simulink model "aerodynamic_model_V1_2_Wrench"  (R2025b)
settings: Solver=ode4  StartTime=0.0  StopTime=0.3  FixedStep=Ts  RelTol=1e-3
InitFcn:
  | % Run initial_main.m first to load Ad,As,Tq_prop,Tq_mass,...
values from neighbouring files (symbols this model uses):
  alpha_du0_v_tail_L = trim_aero_ic.v_tail_L.alpha_du0    [initial_main_V1_1.m]
  alpha_du0_v_tail_R = trim_aero_ic.v_tail_R.alpha_du0    [initial_main_V1_1.m]
  alpha_du0_wing_L = trim_aero_ic.wing_L.alpha_du0    [initial_main_V1_1.m]
  alpha_du0_wing_R = trim_aero_ic.wing_R.alpha_du0    [initial_main_V1_1.m]
  As = sys_sd.A    [initial_main_V1_1.m]
  BladePitch_deg = 34    [initial_main_V1_1.m]
  Bs = sys_sd.B    [initial_main_V1_1.m]
  Cs = sys_sd.C    [initial_main_V1_1.m]
  ctrl_delta_lim_deg = strips.delta_lim_deg    [initial_main_V1_1.m]
  ctrl_map_aileron_L = aero.wing_L.map_aileron(:)    [initial_main_V1_1.m]
  ctrl_map_aileron_R = aero.wing_R.map_aileron(:)    [initial_main_V1_1.m]
  ctrl_map_tail_L = aero.v_tail_L.map_tail(:)    [initial_main_V1_1.m]
  ctrl_map_tail_R = aero.v_tail_R.map_tail(:)    [initial_main_V1_1.m]
  Ds = sys_sd.D    [initial_main_V1_1.m]
  I_cg_b = R_sb * I_cg_m * R_sb.'    [aeroelastic.m]    (also in initial_main_V1_1.m = grav.I_cg_b)
  I_cg_b_inv = R_sb * I_cg_m_inv * R_sb.'    [aeroelastic.m]    (also in initial_main_V1_1.m = grav.I_cg_b_inv)
  m_node = zeros(n_id, 1)    [aeroelastic.m]    (also in generate_pullup_load_cloud.m = evalin('base', 'm_node(:)'); initial_main_V1_1.m = nodal.m_node)
  m_total_kg = evalin('base', 'm_total_kg')    [generate_pullup_load_cloud.m]    (also in initial_main_V1_1.m = grav.m_total_kg)
  n_modes = size(Phi, 2)    [aeroelastic.m]    (also in initial_main_V1_1.m = n_rigid + n_elastic)
  ones_1_tail = ones(1, size(r_cg2ac_b_v_tail_L, 2))    [initial_main_V1_1.m]
  ones_1_wing = ones(1, size(r_cg2ac_b_wing_L, 2))    [initial_main_V1_1.m]
  Phi = evalin('base', 'Phi')    [generate_pullup_load_cloud.m]    (also in initial_main_V1_1.m = strips.Phi)
  polar_alpha_deg = polar.alpha_deg(:).'    [initial_main_V1_1.m]
  polar_CD = polar.CD(:).'    [initial_main_V1_1.m]
  polar_CDp = polar.CDp(:).'    [initial_main_V1_1.m]
  polar_CL = polar.CL(:).'    [initial_main_V1_1.m]
  polar_CM = polar.CM(:).'    [initial_main_V1_1.m]
  r_cg2ac_b_v_tail_L = R_sb * aero.v_tail_L.r_ac_s    [initial_main_V1_1.m]
  r_cg2ac_b_v_tail_R = R_sb * aero.v_tail_R.r_ac_s    [initial_main_V1_1.m]
  r_cg2ac_b_wing_L = R_sb * aero.wing_L.r_ac_s    [initial_main_V1_1.m]
  r_cg2ac_b_wing_R = R_sb * aero.wing_R.r_ac_s    [initial_main_V1_1.m]
  r_cg2kink_b = eng.r_cg2kink_b    [initial_main_V1_1.m]
  r_cg2node_b = aeroelastic.node_arms(nodes, 'R_sb', R_sb).r_cg2node_b    [initial_main_V1_1.m]
  surface_nodes = aeroelastic.surface_load_nodes(nodes)    [initial_main_V1_1.m]
  T_aero2W = aeroelastic.wing_aileron_to_W(strips).T    [initial_main_V1_1.m]
  T_prop2W = load_maps.T_prop2W    [initial_main_V1_1.m]
  Tq_mass = load_maps.Tq_mass    [initial_main_V1_1.m]
  trim_Attitude_rad0 = trim_default.Attitude_rad0    [initial_main_V1_1.m]
  trim_Omega_b0 = trim_default.Omega_b0    [initial_main_V1_1.m]
  trim_Position0 = trim_default.Position0    [initial_main_V1_1.m]
  trim_Velocity_b0 = trim_default.Velocity_b0    [initial_main_V1_1.m]
  Ts = 0.001    [initial_main_V1_1.m]
  U = 55    [initial_main_V1_1.m]
  v_tail_cant_rad = deg2rad(v_tail_cant_deg)    [initial_main_V1_1.m]
  W_mass_g = grav.W_mass    [initial_main_V1_1.m]
  x0_structure = trim_default.x0_structure    [initial_main_V1_1.m]
  x0_wagner_v_tail_L = trim_aero_ic.v_tail_L.x0_wagner    [initial_main_V1_1.m]
  x0_wagner_v_tail_R = trim_aero_ic.v_tail_R.x0_wagner    [initial_main_V1_1.m]
  x0_wagner_wing_L = trim_aero_ic.wing_L.x0_wagner    [initial_main_V1_1.m]
  x0_wagner_wing_R = trim_aero_ic.wing_R.x0_wagner    [initial_main_V1_1.m]
undefined symbols (not defined in the file or in its folder): Ad_v_tail_L, Ad_v_tail_R, Ad_wing_L, Ad_wing_R, Bd_v_tail_L, Bd_v_tail_R, Bd_wing_L, Bd_wing_R, c_over_2U_v_tail_L, c_over_2U_v_tail_R, c_over_2U_wing_L, c_over_2U_wing_R, Cd_v_tail_L, Cd_v_tail_R, Cd_wing_L, Cd_wing_R, Dd_v_tail_L, Dd_v_tail_R, Dd_wing_L, Dd_wing_R, G_du_v_tail_L, G_du_v_tail_R, G_du_wing_L, G_du_wing_R, polar_aileron_alpha_deg, polar_aileron_dCD, polar_aileron_dCL, polar_aileron_dCM, polar_aileron_delta_deg, polar_ruddervator_alpha_deg, polar_ruddervator_dCD, polar_ruddervator_dCL, polar_ruddervator_dCM, polar_ruddervator_delta_deg, qS_strip_v_tail_L, qS_strip_v_tail_R, qS_strip_wing_L, qS_strip_wing_R, qSc_strip_v_tail_L, qSc_strip_v_tail_R, qSc_strip_wing_L, qSc_strip_wing_R, T_m2b_v_tail_L, T_m2b_v_tail_R, T_m2b_wing_L, T_m2b_wing_R, T_m2h_v_tail_L, T_m2h_v_tail_R, T_m2h_wing_L, T_m2h_wing_R, Tq_CM_v_tail_L, Tq_CM_v_tail_R, Tq_CM_wing_L, Tq_CM_wing_R, Tq_D_v_tail_L, Tq_D_v_tail_R, Tq_D_wing_L, Tq_D_wing_R, Tq_v_tail_L, Tq_v_tail_R ... (+2)
libraries: Prop_gryo x12, matrix_library x2
(part 2 of 6)

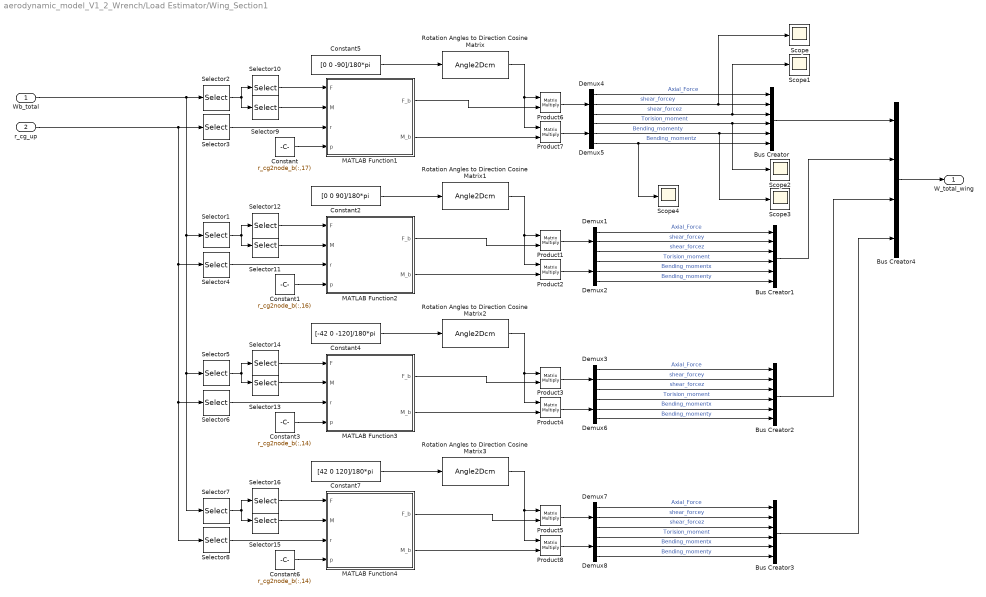
== system aerodynamic_model_V1_2_Wrench/Load Estimator/Wing_Section1 ==
  Wb_total : Inport
  r_cg_up : Inport  Port=2
  Bus Creator{,1..3} (4 alike) : BusCreator  Inputs=6
  Bus Creator4 : BusCreator  Inputs=4
  Constant : Constant  Value=r_cg2node_b(:,17)
  Constant1 : Constant  Value=r_cg2node_b(:,16)
  Constant2 : Constant  Value=[0 0 90]/180*pi
  Constant3 : Constant  Value=r_cg2node_b(:,14)
  Constant4 : Constant  Value=[-42 0 -120]/180*pi
  Constant5 : Constant  Value=[0 0 -90]/180*pi
  Constant6 : Constant  Value=r_cg2node_b(:,14)
  Constant7 : Constant  Value=[42 0 120]/180*pi
  Demux{1..8} (8 alike) : Demux  Outputs=3
  MATLAB Function1 : MATLAB Function  TreatAsAtomicUnit=on
  MATLAB Function2 : MATLAB Function  TreatAsAtomicUnit=on
  MATLAB Function3 : MATLAB Function  TreatAsAtomicUnit=on
  MATLAB Function4 : MATLAB Function  TreatAsAtomicUnit=on
  Product{1..8} (8 alike) : Product  Multiplication=Matrix(*)
  Rotation Angles to Direction Cosine Matrix{,1..3} (4 alike) : Angle2Dcm  rotationOrder=XYZ
      settings: AttributesFormatString=Rotation Order: %<rotationOrder>
  Scope{,1..4} (5 alike) : Scope
      Scope settings: ActiveDisplayYMinimum=-701.70070889117164  ActiveDisplayYMaximum=2692.587568384824  DataLoggingVariableName=ScopeData3
      Scope1 settings: ActiveDisplayYMinimum=-5860.8762190817188  ActiveDisplayYMaximum=-5388.1734134448989  DataLoggingVariableName=ScopeData4
      Scope2 settings: ActiveDisplayYMinimum=-1  ActiveDisplayYMaximum=1  DataLoggingVariableName=ScopeData5
      Scope3 settings: ActiveDisplayYMinimum=-45751.57172735683  ActiveDisplayYMaximum=65131.541259439364  DataLoggingVariableName=ScopeData6
      Scope4 settings: ActiveDisplayYMinimum=-1  ActiveDisplayYMaximum=1  DataLoggingVariableName=ScopeData7
  Selector1 : Selector  NumberOfDimensions=2  InputPortWidth=3  IndexOptions=Select all,Index vector (dialog)  Indices=[1:6],[surface_nodes.wing_R.node_id]  OutputSizes=1,1
  Selector{10,12,14,16} (4 alike) : Selector  NumberOfDimensions=2  InputPortWidth=3  IndexOptions=Index vector (dialog),Select all  Indices=[1:3],[surface_nodes.wing_R.node_id]  OutputSizes=1,1
  Selector{9,11,13,15} (4 alike) : Selector  NumberOfDimensions=2  InputPortWidth=3  IndexOptions=Index vector (dialog),Select all  Indices=[4:6],[surface_nodes.wing_R.node_id]  OutputSizes=1,1
  Selector2 : Selector  NumberOfDimensions=2  InputPortWidth=3  IndexOptions=Select all,Index vector (dialog)  Indices=[1:6],[surface_nodes.wing_L.node_id]  OutputSizes=1,1
  Selector3 : Selector  NumberOfDimensions=2  InputPortWidth=3  IndexOptions=Select all,Index vector (dialog)  Indices=[1:6],[surface_nodes.wing_L.node_id]  OutputSizes=1,1
  Selector4 : Selector  NumberOfDimensions=2  InputPortWidth=3  IndexOptions=Select all,Index vector (dialog)  Indices=[1:6],[surface_nodes.wing_R.node_id]  OutputSizes=1,1
  Selector5 : Selector  NumberOfDimensions=2  InputPortWidth=3  IndexOptions=Select all,Index vector (dialog)  Indices=[1:6],[surface_nodes.v_tail_L.node_id]  OutputSizes=1,1
  Selector6 : Selector  NumberOfDimensions=2  InputPortWidth=3  IndexOptions=Select all,Index vector (dialog)  Indices=[1:6],[surface_nodes.v_tail_L.node_id]  OutputSizes=1,1
  Selector7 : Selector  NumberOfDimensions=2  InputPortWidth=3  IndexOptions=Select all,Index vector (dialog)  Indices=[1:6],[surface_nodes.v_tail_R.node_id]  OutputSizes=1,1
  Selector8 : Selector  NumberOfDimensions=2  InputPortWidth=3  IndexOptions=Select all,Index vector (dialog)  Indices=[1:6],[surface_nodes.v_tail_R.node_id]  OutputSizes=1,1
  W_total_wing : Outport
  wires:
  Selector9/1 -> MATLAB Function1/2(M)
  Selector10/1 -> MATLAB Function1/1(F)
  Selector2/1 -> Selector9/1, Selector10/1
  Constant/1 -> MATLAB Function1/4(p)
  Bus Creator4/1 -> W_total_wing/1
  Bus Creator3/1 -> Bus Creator4/4
  Bus Creator2/1 -> Bus Creator4/3
  Bus Creator1/1 -> Bus Creator4/2
  Bus Creator/1 -> Bus Creator4/1
  Demux7/1 -> Bus Creator3/1  "Axial_Force"
  Demux8/1 -> Bus Creator3/4  "Torision_moment"
  Demux7/2 -> Bus Creator3/2  "shear_forcey"
  Product8/1 -> Demux8/1
  Demux8/2 -> Bus Creator3/5  "Bending_momentx"
  Demux8/3 -> Bus Creator3/6  "Bending_momenty"
  Demux7/3 -> Bus Creator3/3  "shear_forcez"
  Product5/1 -> Demux7/1
  Product3/1 -> Demux3/1
  Product4/1 -> Demux6/1
  Demux3/2 -> Bus Creator2/2  "shear_forcey"
  Demux6/2 -> Bus Creator2/5  "Bending_momentx"
  Demux3/1 -> Bus Creator2/1  "Axial_Force"
  Demux3/3 -> Bus Creator2/3  "shear_forcez"
  Demux6/3 -> Bus Creator2/6  "Bending_momenty"
  Demux6/1 -> Bus Creator2/4  "Torision_moment"
  Demux2/1 -> Bus Creator1/4  "Torision_moment"
  Demux1/3 -> Bus Creator1/3  "shear_forcez"
  Demux2/3 -> Bus Creator1/6  "Bending_momenty"
  Demux1/2 -> Bus Creator1/2  "shear_forcey"
  Demux2/2 -> Bus Creator1/5  "Bending_momentx"
  Demux1/1 -> Bus Creator1/1  "Axial_Force"
  Demux4/1 -> Bus Creator/1  "Axial_Force"
  Demux5/3 -> Bus Creator/6, Scope4/1  "Bending_momentz"
  Demux5/2 -> Bus Creator/5, Scope3/1  "Bending_momenty"
  Demux5/1 -> Bus Creator/4, Scope2/1  "Torision_moment"
  Demux4/3 -> Bus Creator/3, Scope1/1  "shear_forcez"
  Demux4/2 -> Bus Creator/2, Scope/1  "shear_forcey"
  Selector16/1 -> MATLAB Function4/1(F)
  Selector15/1 -> MATLAB Function4/2(M)
  Selector7/1 -> Selector16/1, Selector15/1
  Selector14/1 -> MATLAB Function3/1(F)
  Selector13/1 -> MATLAB Function3/2(M)
  Selector5/1 -> Selector14/1, Selector13/1
  Selector1/1 -> Selector12/1, Selector11/1
  Selector11/1 -> MATLAB Function2/2(M)
  Selector12/1 -> MATLAB Function2/1(F)
  Product2/1 -> Demux2/1
  Product1/1 -> Demux1/1
  Product7/1 -> Demux5/1
  Product6/1 -> Demux4/1
  Constant7/1 -> Rotation Angles to Direction Cosine Matrix3/1
  MATLAB Function4/1(F_b) -> Product5/2
  Selector8/1 -> MATLAB Function4/3(r)
  Constant6/1 -> MATLAB Function4/4(p)
  Rotation Angles to Direction Cosine Matrix3/1 -> Product8/1, Product5/1
  MATLAB Function4/2(M_b) -> Product8/2
  r_cg_up/1 -> Selector3/1, Selector4/1, Selector6/1, Selector8/1
  Wb_total/1 -> Selector2/1, Selector7/1, Selector5/1, Selector1/1
  MATLAB Function3/2(M_b) -> Product4/2
  Rotation Angles to Direction Cosine Matrix2/1 -> Product3/1, Product4/1
  Constant3/1 -> MATLAB Function3/4(p)
  Selector6/1 -> MATLAB Function3/3(r)
  MATLAB Function3/1(F_b) -> Product3/2
  Constant4/1 -> Rotation Angles to Direction Cosine Matrix2/1
  Constant2/1 -> Rotation Angles to Direction Cosine Matrix1/1
  MATLAB Function2/1(F_b) -> Product1/2
  Selector4/1 -> MATLAB Function2/3(r)
  Constant1/1 -> MATLAB Function2/4(p)
  Rotation Angles to Direction Cosine Matrix1/1 -> Product2/1, Product1/1
  MATLAB Function2/2(M_b) -> Product2/2
  MATLAB Function1/2(M_b) -> Product7/2
  Rotation Angles to Direction Cosine Matrix/1 -> Product6/1, Product7/1
  Selector3/1 -> MATLAB Function1/3(r)
  MATLAB Function1/1(F_b) -> Product6/2
  Constant5/1 -> Rotation Angles to Direction Cosine Matrix/1

== system aerodynamic_model_V1_2_Wrench/Propulsion Dynamics/Subsystem8 ==
  In1 : Inport
  In2 : Inport  Port=2
  Vb : Inport  Port=3
  Omegab : Inport  Port=4
  BladePitchAngle_DEG : Inport  Port=5
  RPS : Inport  Port=6
  +Cant : Constant  Value=7/180*pi
  -Cant1 : Constant  Value=-7/180*pi
  -Cant10 : Constant  Value=r_cg2kink_b(:,8)
  -Cant11 : Constant  Value=-0.6
  -Cant2 : Constant  Value=0.6
  -Cant3 : Constant  Value=r_cg2kink_b(:,1)
  -Cant4 : Constant  Value=r_cg2kink_b(:,2)
  -Cant5 : Constant  Value=r_cg2kink_b(:,3)
  -Cant6 : Constant  Value=r_cg2kink_b(:,4)
  -Cant7 : Constant  Value=r_cg2kink_b(:,5)
  -Cant8 : Constant  Value=r_cg2kink_b(:,6)
  -Cant9 : Constant  Value=r_cg2kink_b(:,7)
  Demux : Demux  Outputs=8
  Demux1 : Demux  Outputs=8
  Demux2 : Demux  Outputs=8
  Prop1 : Prop_gryo/Prop1  SystemSampleTime=-1  VariantActivationTime=update diagram  EmptyChoice=off  PassThrough=off  PassThroughVariantControl=(default)  EmptyChoiceVariantControl=(default)  AllowFlexibleInterface=on  Latency=0  AutoFrameSizeCalculation=off
  Prop2 : Prop_gryo/Prop2  SystemSampleTime=-1  VariantActivationTime=update diagram  EmptyChoice=off  PassThrough=off  PassThroughVariantControl=(default)  EmptyChoiceVariantControl=(default)  AllowFlexibleInterface=on  Latency=0  AutoFrameSizeCalculation=off
  Prop3 : Prop_gryo/Prop3  SystemSampleTime=-1  VariantActivationTime=update diagram  EmptyChoice=off  PassThrough=off  PassThroughVariantControl=(default)  EmptyChoiceVariantControl=(default)  AllowFlexibleInterface=on  Latency=0  AutoFrameSizeCalculation=off
  Prop4 : Prop_gryo/Prop4  SystemSampleTime=-1  VariantActivationTime=update diagram  EmptyChoice=off  PassThrough=off  PassThroughVariantControl=(default)  EmptyChoiceVariantControl=(default)  AllowFlexibleInterface=on  Latency=0  AutoFrameSizeCalculation=off
  Prop5 : Prop_gryo/Prop5  SystemSampleTime=-1  VariantActivationTime=update diagram  EmptyChoice=off  PassThrough=off  PassThroughVariantControl=(default)  EmptyChoiceVariantControl=(default)  AllowFlexibleInterface=on  Latency=0  AutoFrameSizeCalculation=off
  Prop6 : Prop_gryo/Prop6  SystemSampleTime=-1  VariantActivationTime=update diagram  EmptyChoice=off  PassThrough=off  PassThroughVariantControl=(default)  EmptyChoiceVariantControl=(default)  AllowFlexibleInterface=on  Latency=0  AutoFrameSizeCalculation=off
  Prop7 : Prop_gryo/Prop7  SystemSampleTime=-1  VariantActivationTime=update diagram  EmptyChoice=off  PassThrough=off  PassThroughVariantControl=(default)  EmptyChoiceVariantControl=(default)  AllowFlexibleInterface=on  Latency=0  AutoFrameSizeCalculation=off
  Prop8 : Prop_gryo/Prop8  SystemSampleTime=-1  VariantActivationTime=update diagram  EmptyChoice=off  PassThrough=off  PassThroughVariantControl=(default)  EmptyChoiceVariantControl=(default)  AllowFlexibleInterface=on  Latency=0  AutoFrameSizeCalculation=off
  Out Bus Element : Outport  PortName=Prop  Element=signal1
  Out Bus Element1 : Outport  PortName=Prop  Element=signal2
  Out Bus Element2 : Outport  PortName=Prop  Element=signal3
  Out Bus Element3 : Outport  PortName=Prop  Element=signal4
  Out Bus Element4 : Outport  PortName=Prop  Element=signal5
  Out Bus Element5 : Outport  PortName=Prop  Element=signal6
  Out Bus Element6 : Outport  PortName=Prop  Element=signal7
  Out Bus Element7 : Outport  PortName=Prop  Element=signal8
  wires:
  In2/1 -> Demux1/1
  -Cant7/1 -> Prop5/4
  Vb/1 -> Prop5/2, Prop1/2, Prop4/2, Prop8/2, Prop7/3, Prop3/3, Prop6/3, Prop2/3
  Demux/7 -> Prop7/2
  Omegab/1 -> Prop5/3, Prop1/3, Prop4/3, Prop8/3, Prop7/4, Prop3/4, Prop6/4, Prop2/4
  Demux1/3 -> Prop3/6
  Demux1/6 -> Prop6/6
  -Cant8/1 -> Prop6/5
  -Cant1/1 -> Prop5/1, Prop1/1, Prop6/1, Prop2/1
  BladePitchAngle_DEG/1 -> Prop6/9, Prop2/9, Prop3/9, Prop7/9
  -Cant6/1 -> Prop4/4
  Demux1/2 -> Prop2/6
  Demux/6 -> Prop6/2
  -Cant5/1 -> Prop3/5
  -Cant4/1 -> Prop2/5
  +Cant/1 -> Prop4/1, Prop8/1, Prop3/1, Prop7/1
  -Cant3/1 -> Prop1/4
  Demux/2 -> Prop2/2
  -Cant10/1 -> Prop8/4
  Demux1/7 -> Prop7/6
  -Cant9/1 -> Prop7/5
  Demux/3 -> Prop3/2
  In1/1 -> Demux/1
  Prop1/1 -> Out Bus Element/1
  Prop2/1 -> Out Bus Element1/1
  RPS/1 -> Demux2/1
  Demux2/1 -> Prop1/6
  Demux2/2 -> Prop2/8
  Demux2/3 -> Prop3/8
  Demux2/4 -> Prop4/6
  Demux2/5 -> Prop5/6
  Demux2/6 -> Prop6/8
  Demux2/7 -> Prop7/8
  Demux2/8 -> Prop8/6
  Prop3/1 -> Out Bus Element2/1
  Prop4/1 -> Out Bus Element3/1
  Prop5/1 -> Out Bus Element4/1
  Prop6/1 -> Out Bus Element5/1
  Prop8/1 -> Out Bus Element7/1
  Prop7/1 -> Out Bus Element6/1
  -Cant2/1 -> Prop2/7, Prop3/7, Prop4/5, Prop1/5
  -Cant11/1 -> Prop6/7, Prop7/7, Prop8/5, Prop5/5

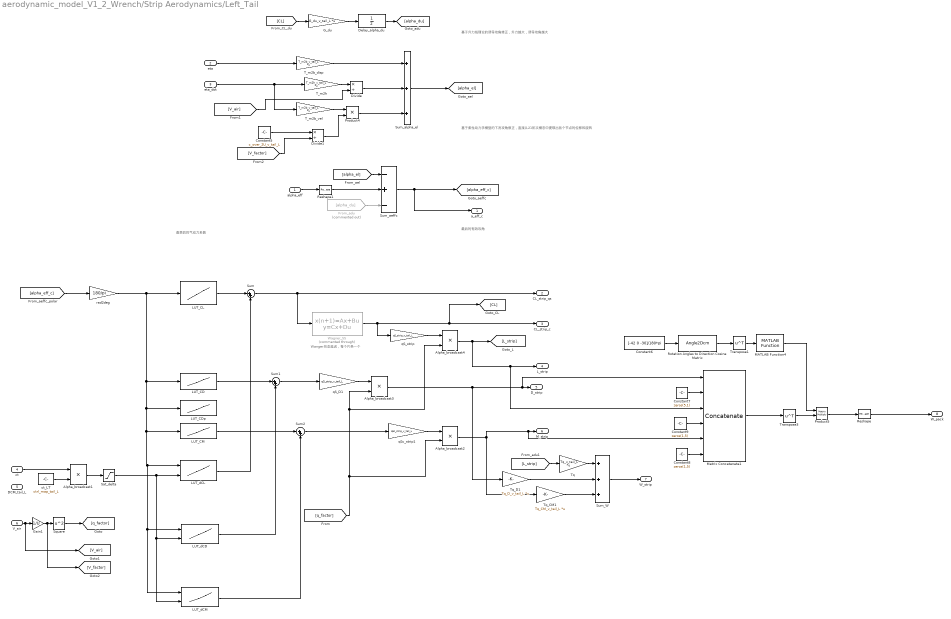
== system aerodynamic_model_V1_2_Wrench/Strip Aerodynamics/Left_Tail ==
  note: 基于升力线理论的诱导攻角修正，升力越大，诱导攻角越大
  note: 基于柔性动力学模型的下洗攻角修正，直接从21阶次模态中提取出各个节点的位移和旋转
  note: 最后的有效攻角
  note: 查表后的气动力系数
  note: Wanger状态延迟，每个片条一个
  alpha_eff : Inport
  eta : Inport  Port=2
  eta_dot : Inport  Port=3
  ct : Inport  Port=4
  DCM_tail_L : Inport  Port=5
  V_air : Inport  Port=6
  Alpha_broadcast{1..4} (4 alike) : Product  Inputs=**
  Constant5 : Constant  Value=c_over_2U_v_tail_L
  Constant6 : Constant  Value=[-42 0 -30]/180*pi
  Constant7 : Constant  Value=zeros(5,1)
  Constant8 : Constant  Value=zeros(1,5)
  Constant9 : Constant  Value=zeros(1,5)
  Delay_alpha_du : UnitDelay  InitialCondition=alpha_du0_v_tail_L  SampleTime=Ts  HasFrameUpgradeWarning=on
  Divide : Product  Inputs=*/
  Divide1 : Product  Inputs=*/
  From_adu : From  Commented=on  GotoTag=alpha_du
  G_du : Gain  Gain=G_du_v_tail_L  Multiplication=Matrix(K*u)
  Gain1 : Gain  Gain=1/U
  LUT_CD : Lookup_n-D  NumberOfTableDimensions=1  BreakpointsForDimension1=polar_alpha_deg  BreakpointsForDimension3=[5, 7]  Table=polar_CD  ExtrapMethod=Clip  InternalRulePriority=Speed  RndMeth=Simplest
  LUT_CDp : Lookup_n-D  NumberOfTableDimensions=1  BreakpointsForDimension1=polar_alpha_deg  BreakpointsForDimension3=[5, 7]  Table=polar_CDp  ExtrapMethod=Clip  InternalRulePriority=Speed  RndMeth=Simplest
  LUT_CL : Lookup_n-D  NumberOfTableDimensions=1  BreakpointsForDimension1=polar_alpha_deg  BreakpointsForDimension3=[5, 7]  Table=polar_CL  ExtrapMethod=Clip  InternalRulePriority=Speed  RndMeth=Simplest
  LUT_CM : Lookup_n-D  NumberOfTableDimensions=1  BreakpointsForDimension1=polar_alpha_deg  BreakpointsForDimension3=[5, 7]  Table=polar_CM  ExtrapMethod=Clip  InternalRulePriority=Speed  RndMeth=Simplest
  LUT_dCD : Lookup_n-D  BreakpointsForDimension1=polar_ruddervator_alpha_deg  BreakpointsForDimension2=polar_ruddervator_delta_deg  BreakpointsForDimension3=[5, 7]  Table=polar_ruddervator_dCD  ExtrapMethod=Clip  InternalRulePriority=Speed  RndMeth=Simplest
      settings: InputPortMap=u0,u1
  LUT_dCL : Lookup_n-D  BreakpointsForDimension1=polar_ruddervator_alpha_deg  BreakpointsForDimension2=polar_ruddervator_delta_deg  BreakpointsForDimension3=[5, 7]  Table=polar_ruddervator_dCL  ExtrapMethod=Clip  InternalRulePriority=Speed  RndMeth=Simplest
      settings: InputPortMap=u0,u1
  LUT_dCM : Lookup_n-D  BreakpointsForDimension1=polar_ruddervator_alpha_deg  BreakpointsForDimension2=polar_ruddervator_delta_deg  BreakpointsForDimension3=[5, 7]  Table=polar_ruddervator_dCM  ExtrapMethod=Clip  InternalRulePriority=Speed  RndMeth=Simplest
      settings: InputPortMap=u0,u1
  MATLAB Function4 : Prop_gryo/Prop1/MATLAB Function  SystemSampleTime=-1  VariantActivationTime=update diagram  EmptyChoice=off  PassThrough=off  PassThroughVariantControl=(default)  EmptyChoiceVariantControl=(default)  AllowFlexibleInterface=on  Latency=0  AutoFrameSizeCalculation=off
  Matrix Concatenate1 : Concatenate  NumInputs=6  Mode=Multidimensional array  ConcatenateDimension=2
  Product4 : Product
  Product5 : Product  Multiplication=Matrix(*)
  Reshape : Reshape
  Reshape1 : Reshape
  Rotation Angles to Direction Cosine Matrix : Angle2Dcm  rotationOrder=XYZ
      settings: AttributesFormatString=Rotation Order: %<rotationOrder>
  Sat_delta : Saturate  UpperLimit=ctrl_delta_lim_deg  LowerLimit=-ctrl_delta_lim_deg
  Square : Math  Operator=square
  Sum : Sum  Inputs=|++
  Sum1 : Sum  Inputs=|++
  Sum2 : Sum  Inputs=|++
  Sum_W : Sum  Inputs=+++
  Sum_aeffc : Sum  Inputs=-+-
  Sum_alpha_el : Sum  Inputs=+++
  T_m2b_disp : Gain  Gain=T_m2b_v_tail_L  Multiplication=Matrix(K*u)
  T_m2b_vel : Gain  Gain=T_m2b_v_tail_L  Multiplication=Matrix(K*u)
  T_m2h : Gain  Gain=T_m2h_v_tail_L  Multiplication=Matrix(K*u)
  Tq : Gain  Gain=Tq_v_tail_L  Multiplication=Matrix(K*u)
  Tq_CM1 : Gain  Gain=Tq_CM_v_tail_L  Multiplication=Matrix(K*u)
  Tq_D1 : Gain  Gain=Tq_D_v_tail_L  Multiplication=Matrix(K*u)
  Transpose1 : Math  Operator=transpose
  Transpose3 : Math  Operator=transpose
  Wagner_SS : DiscreteStateSpace  Commented=through  A=Ad_v_tail_L  B=Bd_v_tail_L  C=Cd_v_tail_L  D=Dd_v_tail_L  InitialCondition=x0_wagner_v_tail_L  SampleTime=Ts
  ct_LT : Constant  Value=ctrl_map_tail_L
  qS_D1 : Gain  Gain=qS_strip_v_tail_L
  qS_strip : Gain  Gain=qS_strip_v_tail_L
  qSc_strip1 : Gain  Gain=qSc_strip_v_tail_L
  rad2deg : Gain  Gain=180/pi
  a_eff_c : Outport
  CL_strip_qs : Outport  Port=2
  CL_strip_c : Outport  Port=3
  L_strip : Outport  Port=4
  D_strip : Outport  Port=5
  M_strip : Outport  Port=6
  W_strip : Outport  Port=7
  W_pack : Outport  Port=8
  wires:
  rad2deg/1 -> LUT_CD/1, LUT_CDp/1, LUT_dCL/1, LUT_dCM/1, LUT_dCD/1, LUT_CM/1, LUT_CL/1
  Wagner_SS/1 -> CL_strip_c/1, [CL], qS_strip/1
  eta/1 -> T_m2b_disp/1
  Delay_alpha_du/1 -> [alpha_du]
  Sum/1 -> CL_strip_qs/1, Wagner_SS/1
  T_m2b_vel/1 -> Product4/1
  Divide/1 -> Sum_alpha_el/2
  T_m2b_disp/1 -> Sum_alpha_el/1
  G_du/1 -> Delay_alpha_du/1
  Product4/1 -> Sum_alpha_el/3
  Sum_alpha_el/1 -> [alpha_el]
  Sum_aeffc/1 -> a_eff_c/1, [alpha_eff_c]
  [alpha_eff_c] -> rad2deg/1
  T_m2h/1 -> Divide/1
  eta_dot/1 -> T_m2b_vel/1, T_m2h/1
  Sum1/1 -> qS_D1/1
  Sum2/1 -> qSc_strip1/1
  [CL] -> G_du/1
  [alpha_el] -> Sum_aeffc/1
  From_adu/1 -> Sum_aeffc/3
  [L_strip] -> Tq/1
  Tq/1 -> Sum_W/1
  Tq_D1/1 -> Sum_W/2
  Tq_CM1/1 -> Sum_W/3
  Sum_W/1 -> W_strip/1
  alpha_eff/1 -> Reshape1/1
  ct/1 -> Alpha_broadcast1/1
  ct_LT/1 -> Alpha_broadcast1/2
  Alpha_broadcast1/1 -> Sat_delta/1
  LUT_CL/1 -> Sum/1
  LUT_dCL/1 -> Sum/2
  LUT_CD/1 -> Sum1/1
  LUT_dCD/1 -> Sum1/2
  LUT_CM/1 -> Sum2/1
  LUT_dCM/1 -> Sum2/2
  Sat_delta/1 -> LUT_dCL/2, LUT_dCM/2, LUT_dCD/2
  Alpha_broadcast4/1 -> Matrix Concatenate1/3, L_strip/1, [L_strip]
  Reshape/1 -> W_pack/1
  Alpha_broadcast3/1 -> Matrix Concatenate1/1, D_strip/1, Tq_D1/1
  Alpha_broadcast2/1 -> Tq_CM1/1, Matrix Concatenate1/5, M_strip/1
  Reshape1/1 -> Sum_aeffc/2
  V_air/1 -> [V_air], Gain1/1
  Square/1 -> [q_factor]
  [q_factor] -> Alpha_broadcast3/2, Alpha_broadcast4/2, Alpha_broadcast2/2
  qSc_strip1/1 -> Alpha_broadcast2/1
  qS_D1/1 -> Alpha_broadcast3/1
  qS_strip/1 -> Alpha_broadcast4/1
  [V_factor] -> Divide1/2
  Constant5/1 -> Divide1/1
  Divide1/1 -> Product4/2
  [V_air] -> Divide/2
  Gain1/1 -> [V_factor], Square/1
  Rotation Angles to Direction Cosine Matrix/1 -> Transpose1/1
  Constant6/1 -> Rotation Angles to Direction Cosine Matrix/1
  Matrix Concatenate1/1 -> Transpose3/1
  Transpose1/1 -> MATLAB Function4/1
  MATLAB Function4/1 -> Product5/1
  Constant7/1 -> Matrix Concatenate1/2
  Constant8/1 -> Matrix Concatenate1/6
  Product5/1 -> Reshape/1
  Transpose3/1 -> Product5/2
  Constant9/1 -> Matrix Concatenate1/4

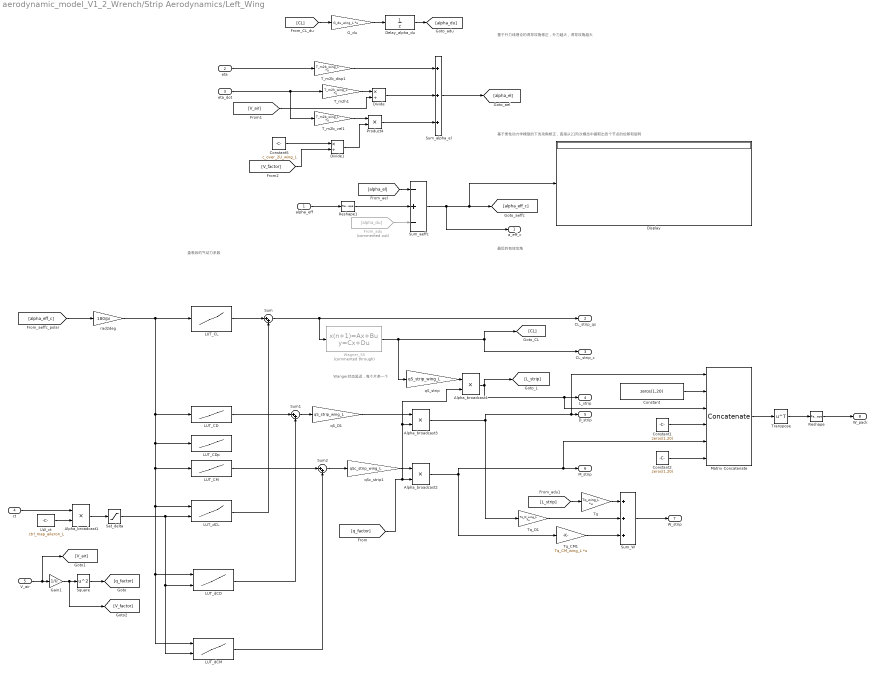
== system aerodynamic_model_V1_2_Wrench/Strip Aerodynamics/Left_Wing ==
  note: 基于升力线理论的诱导攻角修正，升力越大，诱导攻角越大
  note: 基于柔性动力学模型的下洗攻角修正，直接从21阶次模态中提取出各个节点的位移和旋转
  note: 最后的有效攻角
  note: 查表后的气动力系数
  note: Wanger状态延迟，每个片条一个
  alpha_eff : Inport
  eta : Inport  Port=2
  eta_dot : Inport  Port=3
  ct : Inport  Port=4
  V_air : Inport  Port=5
  Alpha_broadcast{1..4} (4 alike) : Product  Inputs=**
  Constant : Constant  Value=zeros(1,20)
  Constant1 : Constant  Value=zeros(1,20)
  Constant2 : Constant  Value=zeros(1,20)
  Constant5 : Constant  Value=c_over_2U_wing_L
  Delay_alpha_du : UnitDelay  InitialCondition=alpha_du0_wing_L  SampleTime=Ts  HasFrameUpgradeWarning=on
  Display : Display
  Divide : Product  Inputs=*/
  Divide1 : Product  Inputs=*/
  From_adu : From  Commented=on  GotoTag=alpha_du
  G_du : Gain  Gain=G_du_wing_L  Multiplication=Matrix(K*u)
  Gain1 : Gain  Gain=1/U
  LUT_CD : Lookup_n-D  NumberOfTableDimensions=1  BreakpointsForDimension1=polar_alpha_deg  BreakpointsForDimension3=[5, 7]  Table=polar_CD  ExtrapMethod=Clip  InternalRulePriority=Speed  RndMeth=Simplest
  LUT_CDp : Lookup_n-D  NumberOfTableDimensions=1  BreakpointsForDimension1=polar_alpha_deg  BreakpointsForDimension3=[5, 7]  Table=polar_CDp  ExtrapMethod=Clip  InternalRulePriority=Speed  RndMeth=Simplest
  LUT_CL : Lookup_n-D  NumberOfTableDimensions=1  BreakpointsForDimension1=polar_alpha_deg  BreakpointsForDimension3=[5, 7]  Table=polar_CL  ExtrapMethod=Clip  InternalRulePriority=Speed  RndMeth=Simplest
  LUT_CM : Lookup_n-D  NumberOfTableDimensions=1  BreakpointsForDimension1=polar_alpha_deg  BreakpointsForDimension3=[5, 7]  Table=polar_CM  ExtrapMethod=Clip  InternalRulePriority=Speed  RndMeth=Simplest
  LUT_dCD : Lookup_n-D  BreakpointsForDimension1=polar_aileron_alpha_deg  BreakpointsForDimension2=polar_aileron_delta_deg  BreakpointsForDimension3=[5, 7]  Table=polar_aileron_dCD  ExtrapMethod=Clip  InternalRulePriority=Speed  RndMeth=Simplest
      settings: InputPortMap=u0,u1
  LUT_dCL : Lookup_n-D  BreakpointsForDimension1=polar_aileron_alpha_deg  BreakpointsForDimension2=polar_aileron_delta_deg  BreakpointsForDimension3=[5, 7]  Table=polar_aileron_dCL  ExtrapMethod=Clip  InternalRulePriority=Speed  RndMeth=Simplest
      settings: InputPortMap=u0,u1
  LUT_dCM : Lookup_n-D  BreakpointsForDimension1=polar_aileron_alpha_deg  BreakpointsForDimension2=polar_aileron_delta_deg  BreakpointsForDimension3=[5, 7]  Table=polar_aileron_dCM  ExtrapMethod=Clip  InternalRulePriority=Speed  RndMeth=Simplest
      settings: InputPortMap=u0,u1
  LW_ct : Constant  Value=ctrl_map_aileron_L
  Matrix Concatenate : Concatenate  NumInputs=6  Mode=Multidimensional array  ConcatenateDimension=2
  Product4 : Product
  Reshape : Reshape
  Reshape1 : Reshape
  Sat_delta : Saturate  UpperLimit=ctrl_delta_lim_deg  LowerLimit=-ctrl_delta_lim_deg
  Square : Math  Operator=square
  Sum : Sum  Inputs=|++
  Sum1 : Sum  Inputs=|++
  Sum2 : Sum  Inputs=|++
  Sum_W : Sum  Inputs=+++
  Sum_aeffc : Sum  Inputs=-+-
  Sum_alpha_el : Sum  Inputs=+++
  T_m2b_disp1 : Gain  Gain=T_m2b_wing_L  Multiplication=Matrix(K*u)
  T_m2b_vel1 : Gain  Gain=T_m2b_wing_L  Multiplication=Matrix(K*u)
  T_m2h1 : Gain  Gain=T_m2h_wing_L  Multiplication=Matrix(K*u)
  Tq : Gain  Gain=Tq_wing_L  Multiplication=Matrix(K*u)
  Tq_CM1 : Gain  Gain=Tq_CM_wing_L  Multiplication=Matrix(K*u)
  Tq_D1 : Gain  Gain=Tq_D_wing_L  Multiplication=Matrix(K*u)
  Transpose : Math  Operator=transpose
  Wagner_SS : DiscreteStateSpace  Commented=through  A=Ad_wing_L  B=Bd_wing_L  C=Cd_wing_L  D=Dd_wing_L  InitialCondition=x0_wagner_wing_L  SampleTime=Ts
  qS_D1 : Gain  Gain=qS_strip_wing_L
  qS_strip : Gain  Gain=qS_strip_wing_L
  qSc_strip1 : Gain  Gain=qSc_strip_wing_L
  rad2deg : Gain  Gain=180/pi
  a_eff_c : Outport
  CL_strip_qs : Outport  Port=2
  CL_strip_c : Outport  Port=3
  L_strip : Outport  Port=4
  D_strip : Outport  Port=5
  M_strip : Outport  Port=6
  W_strip : Outport  Port=7
  W_pack : Outport  Port=8
  wires:
  rad2deg/1 -> LUT_CD/1, LUT_CDp/1, LUT_dCM/1, LUT_dCD/1, LUT_dCL/1, LUT_CM/1, LUT_CL/1
  Wagner_SS/1 -> qS_strip/1, CL_strip_c/1, [CL]
  Delay_alpha_du/1 -> [alpha_du]
  Sum/1 -> CL_strip_qs/1, Wagner_SS/1
  G_du/1 -> Delay_alpha_du/1
  Sum_alpha_el/1 -> [alpha_el]
  Sum_aeffc/1 -> a_eff_c/1, Display/1, [alpha_eff_c]
  [alpha_eff_c] -> rad2deg/1
  Sum1/1 -> qS_D1/1
  Sum2/1 -> qSc_strip1/1
  [CL] -> G_du/1
  [alpha_el] -> Sum_aeffc/1
  From_adu/1 -> Sum_aeffc/3
  Alpha_broadcast2/1 -> Tq_CM1/1, Matrix Concatenate/5, M_strip/1
  [L_strip] -> Tq/1
  Tq/1 -> Sum_W/1
  Tq_D1/1 -> Sum_W/2
  Tq_CM1/1 -> Sum_W/3
  Sum_W/1 -> W_strip/1
  alpha_eff/1 -> Reshape1/1
  ct/1 -> Alpha_broadcast1/1
  LW_ct/1 -> Alpha_broadcast1/2
  Alpha_broadcast1/1 -> Sat_delta/1
  LUT_CL/1 -> Sum/1
  LUT_dCL/1 -> Sum/2
  LUT_CD/1 -> Sum1/1
  LUT_dCD/1 -> Sum1/2
  LUT_CM/1 -> Sum2/1
  LUT_dCM/1 -> Sum2/2
  Sat_delta/1 -> LUT_dCM/2, LUT_dCD/2, LUT_dCL/2
  Alpha_broadcast4/1 -> Matrix Concatenate/3, L_strip/1, [L_strip]
  Alpha_broadcast3/1 -> Tq_D1/1, Matrix Concatenate/1, D_strip/1
  Matrix Concatenate/1 -> Transpose/1
  Transpose/1 -> Reshape/1
  Reshape/1 -> W_pack/1
  Constant/1 -> Matrix Concatenate/2
  Constant1/1 -> Matrix Concatenate/4
  Constant2/1 -> Matrix Concatenate/6
  Reshape1/1 -> Sum_aeffc/2
  V_air/1 -> [V_air], Gain1/1
  Gain1/1 -> [V_factor], Square/1
  Square/1 -> [q_factor]
  qSc_strip1/1 -> Alpha_broadcast2/1
  [q_factor] -> Alpha_broadcast4/2, Alpha_broadcast3/2, Alpha_broadcast2/2
  qS_D1/1 -> Alpha_broadcast3/1
  qS_strip/1 -> Alpha_broadcast4/1
  T_m2b_disp1/1 -> Sum_alpha_el/1
  Product4/1 -> Sum_alpha_el/3
  [V_factor] -> Divide1/2
  Divide/1 -> Sum_alpha_el/2
  Constant5/1 -> Divide1/1
  T_m2h1/1 -> Divide/1
  eta/1 -> T_m2b_disp1/1
  eta_dot/1 -> T_m2b_vel1/1, T_m2h1/1
  Divide1/1 -> Product4/2
  T_m2b_vel1/1 -> Product4/1
  [V_air] -> Divide/2

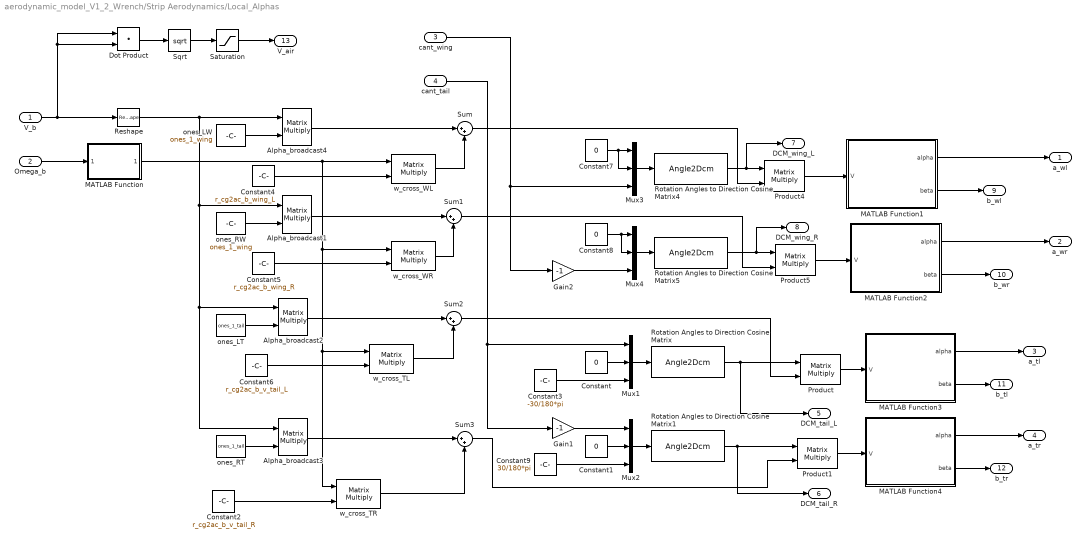
== system aerodynamic_model_V1_2_Wrench/Strip Aerodynamics/Local_Alphas ==
  V_b : Inport  PortDimensions=3
  Omega_b : Inport  Port=2
  cant_wing : Inport  Port=3  PortDimensions=1
  cant_tail : Inport  Port=4
  Alpha_broadcast{1..4} (4 alike) : Product  Multiplication=Matrix(*)
  Constant{,1,7..8} (4 alike) : Constant  Value=0
  Constant2 : Constant  Value=r_cg2ac_b_v_tail_R  VectorParams1D=off
  Constant3 : Constant  Value=-30/180*pi
  Constant4 : Constant  Value=r_cg2ac_b_wing_L  VectorParams1D=off
  Constant5 : Constant  Value=r_cg2ac_b_wing_R  VectorParams1D=off
  Constant6 : Constant  Value=r_cg2ac_b_v_tail_L  VectorParams1D=off
  Constant9 : Constant  Value=30/180*pi
  Dot Product : DotProduct  OutDataTypeStr=Inherit: Inherit via internal rule
  Gain1 : Gain  Gain=-1
  Gain2 : Gain  Gain=-1
  MATLAB Function : MATLAB Function  TreatAsAtomicUnit=on
  MATLAB Function1 : MATLAB Function  TreatAsAtomicUnit=on
  MATLAB Function2 : MATLAB Function  TreatAsAtomicUnit=on
  MATLAB Function3 : MATLAB Function  TreatAsAtomicUnit=on
  MATLAB Function4 : MATLAB Function  TreatAsAtomicUnit=on
  Mux{1..4} (4 alike) : Mux  Inputs=3
  Product{,1,4..5} (4 alike) : Product  Multiplication=Matrix(*)
  Reshape : Reshape  OutputDimensionality=Customize  OutputDimensions=[3 1]
  Rotation Angles to Direction Cosine Matrix{,1,4..5} (4 alike) : Angle2Dcm  rotationOrder=XYZ
      settings: AttributesFormatString=Rotation Order: %<rotationOrder>
  Saturation : Saturate  UpperLimit=inf  LowerLimit=1e-6
  Sqrt : Sqrt
  Sum{,1..3} (4 alike) : Sum  Inputs=|++
  ones_LT : Constant  Value=ones_1_tail  VectorParams1D=off
  ones_LW : Constant  Value=ones_1_wing  VectorParams1D=off
  ones_RT : Constant  Value=ones_1_tail  VectorParams1D=off
  ones_RW : Constant  Value=ones_1_wing  VectorParams1D=off
  w_cross_TL : Product  Multiplication=Matrix(*)
  w_cross_TR : Product  Multiplication=Matrix(*)
  w_cross_WL : Product  Multiplication=Matrix(*)
  w_cross_WR : Product  Multiplication=Matrix(*)
  a_wl : Outport
  a_wr : Outport  Port=2
  a_tl : Outport  Port=3
  a_tr : Outport  Port=4
  DCM_tail_L : Outport  Port=5
  DCM_tail_R : Outport  Port=6
  DCM_wing_L : Outport  Port=7
  DCM_wing_R : Outport  Port=8
  b_wl : Outport  Port=9
  b_wr : Outport  Port=10
  b_tl : Outport  Port=11
  b_tr : Outport  Port=12
  V_air : Outport  Port=13
  wires:
  cant_tail/1 -> Mux1/1, Gain1/1
  Mux1/1 -> Rotation Angles to Direction Cosine Matrix/1
  Mux2/1 -> Rotation Angles to Direction Cosine Matrix1/1
  Constant/1 -> Mux1/2
  Constant1/1 -> Mux2/2
  Rotation Angles to Direction Cosine Matrix/1 -> Product/1, DCM_tail_L/1
  Rotation Angles to Direction Cosine Matrix1/1 -> DCM_tail_R/1, Product1/1
  Product/1 -> MATLAB Function3/1(V)
  Product1/1 -> MATLAB Function4/1(V)
  MATLAB Function1/1(alpha) -> a_wl/1
  MATLAB Function1/2(beta) -> b_wl/1
  Sum/1 -> Product4/2
  ones_LW/1 -> Alpha_broadcast4/2
  Alpha_broadcast4/1 -> Sum/1
  ones_RW/1 -> Alpha_broadcast1/2
  Sum1/1 -> Product5/2
  MATLAB Function2/2(beta) -> b_wr/1
  MATLAB Function2/1(alpha) -> a_wr/1
  ones_LT/1 -> Alpha_broadcast2/2
  Alpha_broadcast2/1 -> Sum2/1
  Mux3/1 -> Rotation Angles to Direction Cosine Matrix4/1
  Constant7/1 -> Mux3/2, Mux3/1
  Constant8/1 -> Mux4/2, Mux4/1
  cant_wing/1 -> Mux3/3, Gain2/1
  Mux4/1 -> Rotation Angles to Direction Cosine Matrix5/1
  Rotation Angles to Direction Cosine Matrix4/1 -> DCM_wing_L/1, Product4/1
  Product4/1 -> MATLAB Function1/1(V)
  Product5/1 -> MATLAB Function2/1(V)
  Rotation Angles to Direction Cosine Matrix5/1 -> DCM_wing_R/1, Product5/1
  Alpha_broadcast3/1 -> Sum3/1
  ones_RT/1 -> Alpha_broadcast3/2
  Reshape/1 -> Alpha_broadcast4/1, Alpha_broadcast3/1, Alpha_broadcast2/1, Alpha_broadcast1/1
  Sum2/1 -> Product/2
  Sum3/1 -> Product1/2
  MATLAB Function3/1(alpha) -> a_tl/1
  MATLAB Function4/1(alpha) -> a_tr/1
  MATLAB Function3/2(beta) -> b_tl/1
  MATLAB Function4/2(beta) -> b_tr/1
  Alpha_broadcast1/1 -> Sum1/1
  V_b/1 -> Dot Product/2, Dot Product/1, Reshape/1
  Omega_b/1 -> MATLAB Function/1(omega)
  MATLAB Function/1(Omega_skew) -> w_cross_TL/1, w_cross_TR/1, w_cross_WR/1, w_cross_WL/1
  Constant4/1 -> w_cross_WL/2
  w_cross_WL/1 -> Sum/2
  Constant5/1 -> w_cross_WR/2
  w_cross_WR/1 -> Sum1/2
  Constant6/1 -> w_cross_TL/2
  w_cross_TL/1 -> Sum2/2
  Constant2/1 -> w_cross_TR/2
  w_cross_TR/1 -> Sum3/2
  Dot Product/1 -> Sqrt/1
  Sqrt/1 -> Saturation/1
  Saturation/1 -> V_air/1
  Gain2/1 -> Mux4/3
  Gain1/1 -> Mux2/1
  Constant3/1 -> Mux1/3
  Constant9/1 -> Mux2/3

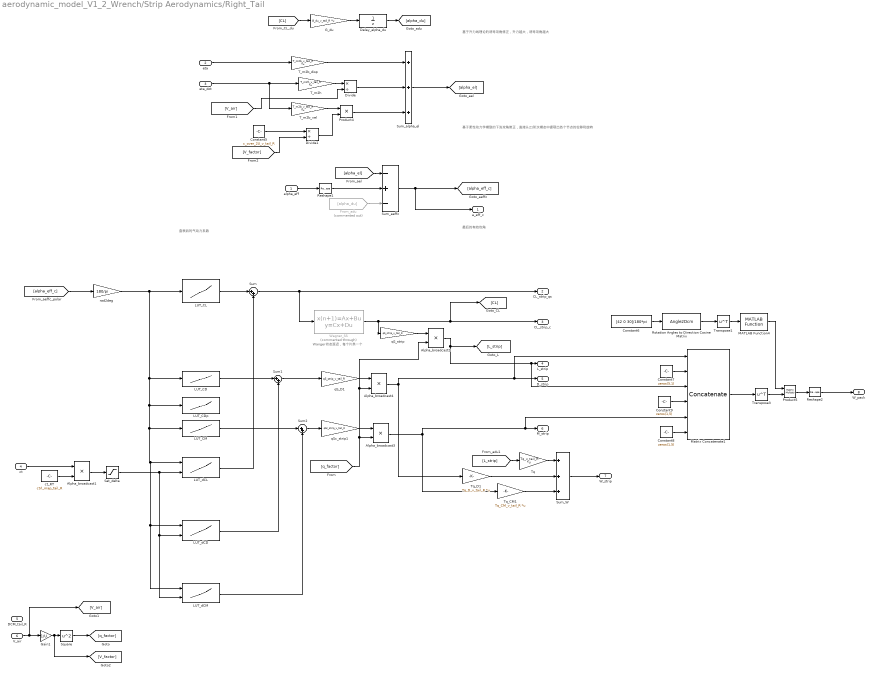
== system aerodynamic_model_V1_2_Wrench/Strip Aerodynamics/Right_Tail ==
  note: Wanger状态延迟，每个片条一个
  note: 查表后的气动力系数
  note: 最后的有效攻角
  note: 基于柔性动力学模型的下洗攻角修正，直接从21阶次模态中提取出各个节点的位移和旋转
  note: 基于升力线理论的诱导攻角修正，升力越大，诱导攻角越大
  alpha_eff : Inport
  eta : Inport  Port=2
  eta_dot : Inport  Port=3
  ct : Inport  Port=4
  DCM_tail_R : Inport  Port=5
  V_air : Inport  Port=6
  Alpha_broadcast{1..4} (4 alike) : Product  Inputs=**
  Constant5 : Constant  Value=c_over_2U_v_tail_R
  Constant6 : Constant  Value=[42 0 30]/180*pi
  Constant7 : Constant  Value=zeros(5,1)
  Constant8 : Constant  Value=zeros(1,5)
  Constant9 : Constant  Value=zeros(1,5)
  Delay_alpha_du : UnitDelay  InitialCondition=alpha_du0_v_tail_R  SampleTime=Ts  HasFrameUpgradeWarning=on
  Divide : Product  Inputs=*/
  Divide1 : Product  Inputs=*/
  From_adu : From  Commented=on  GotoTag=alpha_du
  G_du : Gain  Gain=G_du_v_tail_R  Multiplication=Matrix(K*u)
  Gain1 : Gain  Gain=1/U
  LUT_CD : Lookup_n-D  NumberOfTableDimensions=1  BreakpointsForDimension1=polar_alpha_deg  BreakpointsForDimension3=[5, 7]  Table=polar_CD  ExtrapMethod=Clip  InternalRulePriority=Speed  RndMeth=Simplest
  LUT_CDp : Lookup_n-D  NumberOfTableDimensions=1  BreakpointsForDimension1=polar_alpha_deg  BreakpointsForDimension3=[5, 7]  Table=polar_CDp  ExtrapMethod=Clip  InternalRulePriority=Speed  RndMeth=Simplest
  LUT_CL : Lookup_n-D  NumberOfTableDimensions=1  BreakpointsForDimension1=polar_alpha_deg  BreakpointsForDimension3=[5, 7]  Table=polar_CL  ExtrapMethod=Clip  InternalRulePriority=Speed  RndMeth=Simplest
  LUT_CM : Lookup_n-D  NumberOfTableDimensions=1  BreakpointsForDimension1=polar_alpha_deg  BreakpointsForDimension3=[5, 7]  Table=polar_CM  ExtrapMethod=Clip  InternalRulePriority=Speed  RndMeth=Simplest
  LUT_dCD : Lookup_n-D  BreakpointsForDimension1=polar_ruddervator_alpha_deg  BreakpointsForDimension2=polar_ruddervator_delta_deg  BreakpointsForDimension3=[5, 7]  Table=polar_ruddervator_dCD  ExtrapMethod=Clip  InternalRulePriority=Speed  RndMeth=Simplest
      settings: InputPortMap=u0,u1
  LUT_dCL : Lookup_n-D  BreakpointsForDimension1=polar_ruddervator_alpha_deg  BreakpointsForDimension2=polar_ruddervator_delta_deg  BreakpointsForDimension3=[5, 7]  Table=polar_ruddervator_dCL  ExtrapMethod=Clip  InternalRulePriority=Speed  RndMeth=Simplest
      settings: InputPortMap=u0,u1
  LUT_dCM : Lookup_n-D  BreakpointsForDimension1=polar_ruddervator_alpha_deg  BreakpointsForDimension2=polar_ruddervator_delta_deg  BreakpointsForDimension3=[5, 7]  Table=polar_ruddervator_dCM  ExtrapMethod=Clip  InternalRulePriority=Speed  RndMeth=Simplest
      settings: InputPortMap=u0,u1
  MATLAB Function4 : Prop_gryo/Prop1/MATLAB Function  SystemSampleTime=-1  VariantActivationTime=update diagram  EmptyChoice=off  PassThrough=off  PassThroughVariantControl=(default)  EmptyChoiceVariantControl=(default)  AllowFlexibleInterface=on  Latency=0  AutoFrameSizeCalculation=off
  Matrix Concatenate1 : Concatenate  NumInputs=6  Mode=Multidimensional array  ConcatenateDimension=2
  Product4 : Product
  Product5 : Product  Multiplication=Matrix(*)
  Reshape1 : Reshape
  Reshape2 : Reshape
  Rotation Angles to Direction Cosine Matrix : Angle2Dcm  rotationOrder=XYZ
      settings: AttributesFormatString=Rotation Order: %<rotationOrder>
  Sat_delta : Saturate  UpperLimit=ctrl_delta_lim_deg  LowerLimit=-ctrl_delta_lim_deg
  Square : Math  Operator=square
  Sum : Sum  Inputs=|++
  Sum1 : Sum  Inputs=|++
  Sum2 : Sum  Inputs=|++
  Sum_W : Sum  Inputs=+++
  Sum_aeffc : Sum  Inputs=-+-
  Sum_alpha_el : Sum  Inputs=+++
  T_m2b_disp : Gain  Gain=T_m2b_v_tail_R  Multiplication=Matrix(K*u)
  T_m2b_vel : Gain  Gain=T_m2b_v_tail_R  Multiplication=Matrix(K*u)
  T_m2h : Gain  Gain=T_m2h_v_tail_R  Multiplication=Matrix(K*u)
  Tq : Gain  Gain=Tq_v_tail_R  Multiplication=Matrix(K*u)
  Tq_CM1 : Gain  Gain=Tq_CM_v_tail_R  Multiplication=Matrix(K*u)
  Tq_D1 : Gain  Gain=Tq_D_v_tail_R  Multiplication=Matrix(K*u)
  Transpose1 : Math  Operator=transpose
  Transpose3 : Math  Operator=transpose
  Wagner_SS : DiscreteStateSpace  Commented=through  A=Ad_v_tail_R  B=Bd_v_tail_R  C=Cd_v_tail_R  D=Dd_v_tail_R  InitialCondition=x0_wagner_v_tail_R  SampleTime=Ts
  ct_RT : Constant  Value=ctrl_map_tail_R
  qS_D1 : Gain  Gain=qS_strip_v_tail_R
  qS_strip : Gain  Gain=qS_strip_v_tail_R
  qSc_strip1 : Gain  Gain=qSc_strip_v_tail_R
  rad2deg : Gain  Gain=180/pi
  a_eff_c : Outport
  CL_strip_qs : Outport  Port=2
  CL_strip_c : Outport  Port=3
  L_strip : Outport  Port=4
  D_strip : Outport  Port=5
  M_strip : Outport  Port=6
  W_strip : Outport  Port=7
  W_pack : Outport  Port=8
  wires:
  Sat_delta/1 -> LUT_dCL/2, LUT_dCM/2, LUT_dCD/2
  LUT_dCM/1 -> Sum2/2
  LUT_CM/1 -> Sum2/1
  LUT_dCD/1 -> Sum1/2
  LUT_CD/1 -> Sum1/1
  LUT_dCL/1 -> Sum/2
  LUT_CL/1 -> Sum/1
  Alpha_broadcast1/1 -> Sat_delta/1
  ct_RT/1 -> Alpha_broadcast1/2
  ct/1 -> Alpha_broadcast1/1
  alpha_eff/1 -> Reshape1/1
  Sum_W/1 -> W_strip/1
  Tq_CM1/1 -> Sum_W/3
  Tq_D1/1 -> Sum_W/2
  Tq/1 -> Sum_W/1
  [L_strip] -> Tq/1
  From_adu/1 -> Sum_aeffc/3
  [alpha_el] -> Sum_aeffc/1
  [CL] -> G_du/1
  Sum2/1 -> qSc_strip1/1
  Sum1/1 -> qS_D1/1
  [alpha_eff_c] -> rad2deg/1
  Sum_aeffc/1 -> [alpha_eff_c], a_eff_c/1
  Sum_alpha_el/1 -> [alpha_el]
  G_du/1 -> Delay_alpha_du/1
  Sum/1 -> Wagner_SS/1, CL_strip_qs/1
  Delay_alpha_du/1 -> [alpha_du]
  Wagner_SS/1 -> qS_strip/1, [CL], CL_strip_c/1
  rad2deg/1 -> LUT_CL/1, LUT_CM/1, LUT_dCL/1, LUT_dCM/1, LUT_dCD/1, LUT_CDp/1, LUT_CD/1
  Alpha_broadcast4/1 -> Matrix Concatenate1/1, D_strip/1, Tq_D1/1
  Alpha_broadcast2/1 -> Matrix Concatenate1/3, L_strip/1, [L_strip]
  Alpha_broadcast3/1 -> Tq_CM1/1, Matrix Concatenate1/5, M_strip/1
  Reshape1/1 -> Sum_aeffc/2
  Square/1 -> [q_factor]
  V_air/1 -> [V_air], Gain1/1
  [q_factor] -> Alpha_broadcast2/2, Alpha_broadcast4/2, Alpha_broadcast3/2
  qSc_strip1/1 -> Alpha_broadcast3/1
  qS_D1/1 -> Alpha_broadcast4/1
  qS_strip/1 -> Alpha_broadcast2/1
  [V_factor] -> Divide1/2
  Divide1/1 -> Product4/2
  T_m2h/1 -> Divide/1
  T_m2b_vel/1 -> Product4/1
  eta_dot/1 -> T_m2b_vel/1, T_m2h/1
  eta/1 -> T_m2b_disp/1
  Constant5/1 -> Divide1/1
  T_m2b_disp/1 -> Sum_alpha_el/1
  Divide/1 -> Sum_alpha_el/2
  Product4/1 -> Sum_alpha_el/3
  [V_air] -> Divide/2
  Gain1/1 -> [V_factor], Square/1
  Product5/1 -> Reshape2/1
  Constant8/1 -> Matrix Concatenate1/6
  Transpose1/1 -> MATLAB Function4/1
  MATLAB Function4/1 -> Product5/1
  Rotation Angles to Direction Cosine Matrix/1 -> Transpose1/1
  Reshape2/1 -> W_pack/1
  Constant7/1 -> Matrix Concatenate1/2
  Transpose3/1 -> Product5/2
  Constant9/1 -> Matrix Concatenate1/4
  Constant6/1 -> Rotation Angles to Direction Cosine Matrix/1
  Matrix Concatenate1/1 -> Transpose3/1

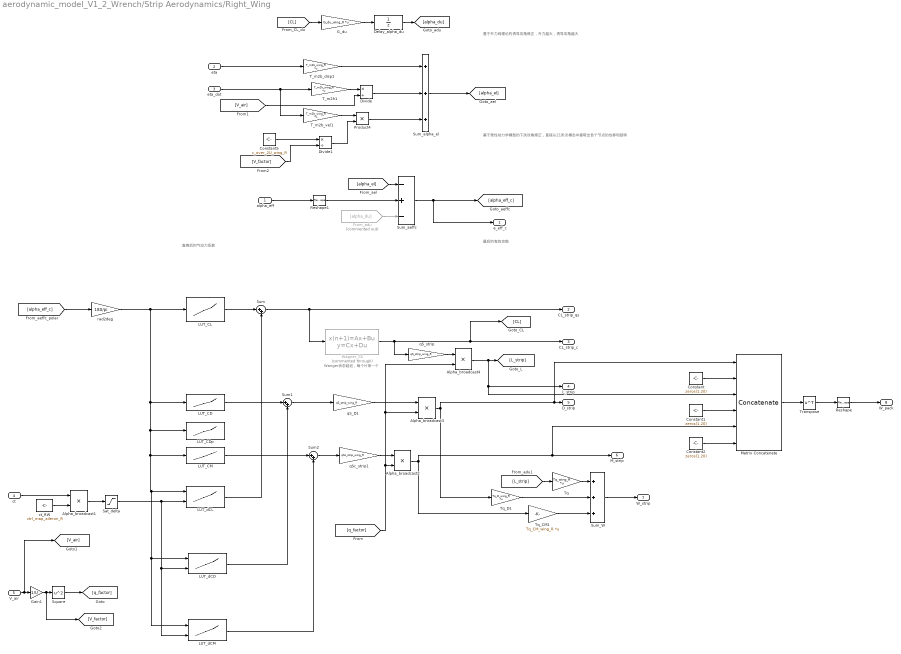
== system aerodynamic_model_V1_2_Wrench/Strip Aerodynamics/Right_Wing ==
  note: Wanger状态延迟，每个片条一个
  note: 查表后的气动力系数
  note: 最后的有效攻角
  note: 基于柔性动力学模型的下洗攻角修正，直接从21阶次模态中提取出各个节点的位移和旋转
  note: 基于升力线理论的诱导攻角修正，升力越大，诱导攻角越大
  alpha_eff : Inport
  eta : Inport  Port=2
  eta_dot : Inport  Port=3
  ct : Inport  Port=4
  V_air : Inport  Port=5
  Alpha_broadcast{1..4} (4 alike) : Product  Inputs=**
  Constant : Constant  Value=zeros(1,20)
  Constant1 : Constant  Value=zeros(1,20)
  Constant2 : Constant  Value=zeros(1,20)
  Constant5 : Constant  Value=c_over_2U_wing_R
  Delay_alpha_du : UnitDelay  InitialCondition=alpha_du0_wing_R  SampleTime=Ts  HasFrameUpgradeWarning=on
  Divide : Product  Inputs=*/
  Divide1 : Product  Inputs=*/
  From_adu : From  Commented=on  GotoTag=alpha_du
  G_du : Gain  Gain=G_du_wing_R  Multiplication=Matrix(K*u)
  Gain1 : Gain  Gain=1/U
  LUT_CD : Lookup_n-D  NumberOfTableDimensions=1  BreakpointsForDimension1=polar_alpha_deg  BreakpointsForDimension3=[5, 7]  Table=polar_CD  ExtrapMethod=Clip  InternalRulePriority=Speed  RndMeth=Simplest
  LUT_CDp : Lookup_n-D  NumberOfTableDimensions=1  BreakpointsForDimension1=polar_alpha_deg  BreakpointsForDimension3=[5, 7]  Table=polar_CDp  ExtrapMethod=Clip  InternalRulePriority=Speed  RndMeth=Simplest
  LUT_CL : Lookup_n-D  NumberOfTableDimensions=1  BreakpointsForDimension1=polar_alpha_deg  BreakpointsForDimension3=[5, 7]  Table=polar_CL  ExtrapMethod=Clip  InternalRulePriority=Speed  RndMeth=Simplest
  LUT_CM : Lookup_n-D  NumberOfTableDimensions=1  BreakpointsForDimension1=polar_alpha_deg  BreakpointsForDimension3=[5, 7]  Table=polar_CM  ExtrapMethod=Clip  InternalRulePriority=Speed  RndMeth=Simplest
  LUT_dCD : Lookup_n-D  BreakpointsForDimension1=polar_aileron_alpha_deg  BreakpointsForDimension2=polar_aileron_delta_deg  BreakpointsForDimension3=[5, 7]  Table=polar_aileron_dCD  ExtrapMethod=Clip  InternalRulePriority=Speed  RndMeth=Simplest
      settings: InputPortMap=u0,u1
  LUT_dCL : Lookup_n-D  BreakpointsForDimension1=polar_aileron_alpha_deg  BreakpointsForDimension2=polar_aileron_delta_deg  BreakpointsForDimension3=[5, 7]  Table=polar_aileron_dCL  ExtrapMethod=Clip  InternalRulePriority=Speed  RndMeth=Simplest
      settings: InputPortMap=u0,u1
  LUT_dCM : Lookup_n-D  BreakpointsForDimension1=polar_aileron_alpha_deg  BreakpointsForDimension2=polar_aileron_delta_deg  BreakpointsForDimension3=[5, 7]  Table=polar_aileron_dCM  ExtrapMethod=Clip  InternalRulePriority=Speed  RndMeth=Simplest
      settings: InputPortMap=u0,u1
  Matrix Concatenate : Concatenate  NumInputs=6  Mode=Multidimensional array  ConcatenateDimension=2
  Product4 : Product
  Reshape : Reshape
  Reshape1 : Reshape
  Sat_delta : Saturate  UpperLimit=ctrl_delta_lim_deg  LowerLimit=-ctrl_delta_lim_deg
  Square : Math  Operator=square
  Sum : Sum  Inputs=|++
  Sum1 : Sum  Inputs=|++
  Sum2 : Sum  Inputs=|++
  Sum_W : Sum  Inputs=+++
  Sum_aeffc : Sum  Inputs=-+-
  Sum_alpha_el : Sum  Inputs=+++
  T_m2b_disp1 : Gain  Gain=T_m2b_wing_R  Multiplication=Matrix(K*u)
  T_m2b_vel1 : Gain  Gain=T_m2b_wing_R  Multiplication=Matrix(K*u)
  T_m2h1 : Gain  Gain=T_m2h_wing_R  Multiplication=Matrix(K*u)
  Tq : Gain  Gain=Tq_wing_R  Multiplication=Matrix(K*u)
  Tq_CM1 : Gain  Gain=Tq_CM_wing_R  Multiplication=Matrix(K*u)
  Tq_D1 : Gain  Gain=Tq_D_wing_R  Multiplication=Matrix(K*u)
  Transpose : Math  Operator=transpose
  Wagner_SS : DiscreteStateSpace  Commented=through  A=Ad_wing_R  B=Bd_wing_R  C=Cd_wing_R  D=Dd_wing_R  InitialCondition=x0_wagner_wing_R  SampleTime=Ts
  ct_RW : Constant  Value=ctrl_map_aileron_R
  qS_D1 : Gain  Gain=qS_strip_wing_R
  qS_strip : Gain  Gain=qS_strip_wing_R
  qSc_strip1 : Gain  Gain=qSc_strip_wing_R
  rad2deg : Gain  Gain=180/pi
  a_eff_c : Outport
  CL_strip_qs : Outport  Port=2
  CL_strip_c : Outport  Port=3
  L_strip : Outport  Port=4
  D_strip : Outport  Port=5
  M_strip : Outport  Port=6
  W_strip : Outport  Port=7
  W_pack : Outport  Port=8
  wires:
  Sat_delta/1 -> LUT_dCL/2, LUT_dCD/2, LUT_dCM/2
  LUT_dCM/1 -> Sum2/2
  LUT_CM/1 -> Sum2/1
  LUT_dCD/1 -> Sum1/2
  LUT_CD/1 -> Sum1/1
  LUT_dCL/1 -> Sum/2
  LUT_CL/1 -> Sum/1
  Alpha_broadcast1/1 -> Sat_delta/1
  ct_RW/1 -> Alpha_broadcast1/2
  ct/1 -> Alpha_broadcast1/1
  alpha_eff/1 -> Reshape1/1
  Sum_W/1 -> W_strip/1
  Tq_CM1/1 -> Sum_W/3
  Tq_D1/1 -> Sum_W/2
  Tq/1 -> Sum_W/1
  [L_strip] -> Tq/1
  From_adu/1 -> Sum_aeffc/3
  [alpha_el] -> Sum_aeffc/1
  [CL] -> G_du/1
  Sum2/1 -> qSc_strip1/1
  Sum1/1 -> qS_D1/1
  [alpha_eff_c] -> rad2deg/1
  Sum_aeffc/1 -> [alpha_eff_c], a_eff_c/1
  Sum_alpha_el/1 -> [alpha_el]
  G_du/1 -> Delay_alpha_du/1
  Sum/1 -> Wagner_SS/1, CL_strip_qs/1
  Delay_alpha_du/1 -> [alpha_du]
  Wagner_SS/1 -> qS_strip/1, [CL], CL_strip_c/1
  rad2deg/1 -> LUT_CL/1, LUT_CM/1, LUT_dCL/1, LUT_dCD/1, LUT_dCM/1, LUT_CDp/1, LUT_CD/1
  Alpha_broadcast4/1 -> L_strip/1, Matrix Concatenate/3, [L_strip]
  Transpose/1 -> Reshape/1
  Reshape/1 -> W_pack/1
  Alpha_broadcast2/1 -> Tq_CM1/1, Matrix Concatenate/5, M_strip/1
  Alpha_broadcast3/1 -> Matrix Concatenate/1, D_strip/1, Tq_D1/1
  Matrix Concatenate/1 -> Transpose/1
  Constant/1 -> Matrix Concatenate/2
  Constant1/1 -> Matrix Concatenate/4
  Constant2/1 -> Matrix Concatenate/6
  Reshape1/1 -> Sum_aeffc/2
  V_air/1 -> [V_air], Gain1/1
  Square/1 -> [q_factor]
  [q_factor] -> Alpha_broadcast4/2, Alpha_broadcast3/2, Alpha_broadcast2/2
  qSc_strip1/1 -> Alpha_broadcast2/1
  qS_D1/1 -> Alpha_broadcast3/1
  qS_strip/1 -> Alpha_broadcast4/1
  [V_factor] -> Divide1/2
  Divide1/1 -> Product4/2
  T_m2h1/1 -> Divide/1
  Product4/1 -> Sum_alpha_el/3
  T_m2b_vel1/1 -> Product4/1
  T_m2b_disp1/1 -> Sum_alpha_el/1
  eta_dot/1 -> T_m2b_vel1/1, T_m2h1/1
  eta/1 -> T_m2b_disp1/1
  Divide/1 -> Sum_alpha_el/2
  Constant5/1 -> Divide1/1
  [V_air] -> Divide/2
  Gain1/1 -> [V_factor], Square/1
